simulink model "phase1_tmp36_faults_FaultModel"  (R2026a)
settings: Solver=VariableStepAuto  StopTime=60  EnableMultiTasking=on
settings Model: Creator=vedant  LastModifiedBy=vedant
settings DebuggingCC: InheritedTsInSrcMsg=none

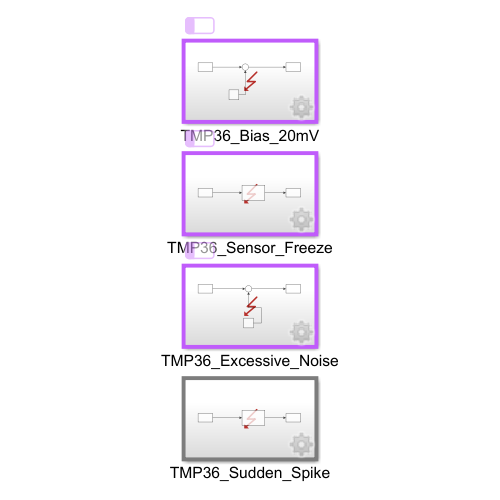
[thumbnail: Simulink's stored preview of the top-level diagram]
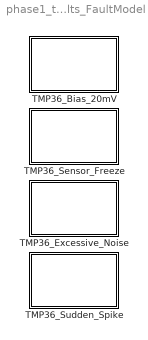
== system phase1_tmp36_faults_FaultModel ==
  TMP36_Bias_20mV : Subsystem  TreatAsAtomicUnit=on  ScheduleAs=Aperiodic partition  PartitionName=PartitionFor_TMP36_Bias_20mV_4022_007690  IsInjectorSS=on
  TMP36_Excessive_Noise : Subsystem  TreatAsAtomicUnit=on  ScheduleAs=Aperiodic partition  PartitionName=PartitionFor_TMP36_Excessive_Noise_4036_005493  IsInjectorSS=on
  TMP36_Sensor_Freeze : Subsystem  TreatAsAtomicUnit=on  ScheduleAs=Aperiodic partition  PartitionName=PartitionFor_TMP36_Sensor_Freeze_4074_003174  IsInjectorSS=on
  TMP36_Sudden_Spike : Subsystem  TreatAsAtomicUnit=on  IsInjectorSS=on

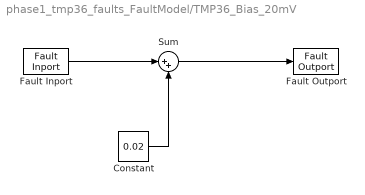
== system phase1_tmp36_faults_FaultModel/TMP36_Bias_20mV ==
  Constant : Constant  Value=0.02
  Fault Inport : FaultInport
  Fault Outport : FaultOutport
  Sum : Sum  Inputs=|++
  wires:
  Fault Inport/1 -> Sum/1
  Sum/1 -> Fault Outport/1
  Constant/1 -> Sum/2

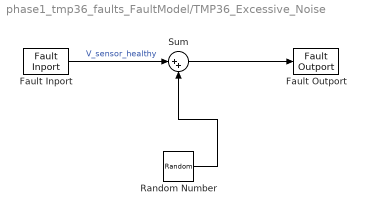
== system phase1_tmp36_faults_FaultModel/TMP36_Excessive_Noise ==
  Fault Inport : FaultInport
  Fault Outport : FaultOutport
  Random Number : RandomNumber  Variance=0.0001  Seed=12345
  Sum : Sum  Inputs=|++
  wires:
  Random Number/1 -> Sum/2
  Fault Inport/1 -> Sum/1  "V_sensor_healthy"
  Sum/1 -> Fault Outport/1

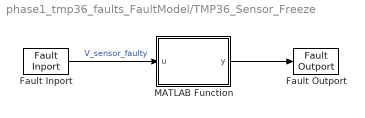
== system phase1_tmp36_faults_FaultModel/TMP36_Sensor_Freeze ==
  Fault Inport : FaultInport
  Fault Outport : FaultOutport
  MATLAB Function : MATLAB Function  TreatAsAtomicUnit=on
  wires:
  Fault Inport/1 -> MATLAB Function/1(u)  "V_sensor_faulty"
  MATLAB Function/1(y) -> Fault Outport/1

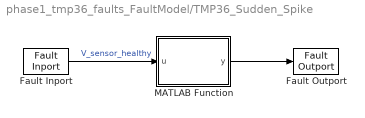
== system phase1_tmp36_faults_FaultModel/TMP36_Sudden_Spike ==
  Fault Inport : FaultInport
  Fault Outport : FaultOutport
  MATLAB Function : MATLAB Function  TreatAsAtomicUnit=on
  wires:
  Fault Inport/1 -> MATLAB Function/1(u)  "V_sensor_healthy"
  MATLAB Function/1(y) -> Fault Outport/1

== matlab function phase1_tmp36_faults_FaultModel/TMP36_Sensor_Freeze/MATLAB Function ==
  data: u input; y output
function y = freezeFault(u)

persistent frozenValue

if isempty(frozenValue)
    frozenValue = u;
end

y = frozenValue;

== matlab function phase1_tmp36_faults_FaultModel/TMP36_Sudden_Spike/MATLAB Function ==
  data: u input; y output
function y = spikeFault(u)

persistent done

if isempty(done)
    done = false;
end

if ~done
    y = u + 0.10;
    done = true;
else
    y = u;
end
